simulink model "gnc_CommandShaping"  (R2026b)
settings: Solver=VariableStepAuto
values from neighbouring files (symbols this model uses):
  Ts = prm.Ts    [gnc_missionFSM.m]    (also in gnc_mpcPlantUpdate.m)
undefined symbols (not defined in the file or in its folder): accel_limit, beacon_cmd, buzzer_cmd, cmd_valid, gnc_ready, gnc_state, GncModeReq, mode_req, nav_fix, omega_cmd, P, seq, soft_stop_req, t_stamp, v_cmd, v_ground_est, v_ground_valid
libraries: simulink x4, sl_discontinuities x1
settings Model: Creator=aomar  LastModifiedBy=aomar

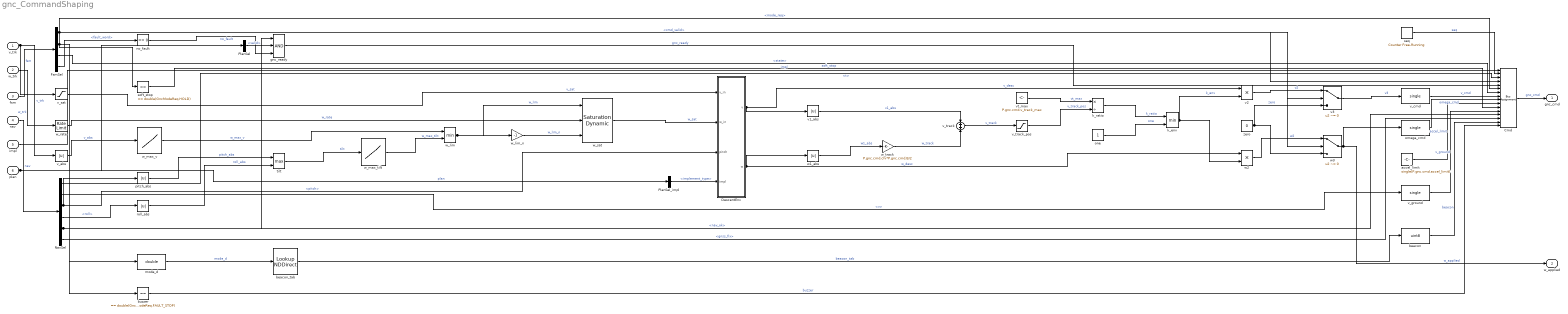
== system gnc_CommandShaping ==
  v_trk : Inport  OutDataTypeStr=double  PortDimensions=1  SampleTime=Ts.gnc
  w_trk : Inport  Port=2  OutDataTypeStr=double  PortDimensions=1  SampleTime=Ts.gnc
  fsm : Inport  Port=3  OutDataTypeStr=Bus: Bus_FsmOut  SampleTime=Ts.gnc
  nav : Inport  Port=4  OutDataTypeStr=Bus: Bus_NavCond  SampleTime=Ts.gnc
  impl : Inport  Port=5  OutDataTypeStr=Bus: Bus_GncCmd  SampleTime=Ts.gnc
  plan : Inport  Port=6  OutDataTypeStr=Bus: Bus_MissionPlan
  Cmd : BusAssignment  AssignedSignals=seq,t_stamp,cmd_valid,gnc_ready,mode_req,gnc_state,v_cmd,omega_cmd,accel_limit,soft_stop_req,v_ground_est,v_ground_valid,nav_fix,beacon_cmd,buzzer_cmd
  DescentEnv : MATLAB Function  TreatAsAtomicUnit=on  mask{desc=P.gnc.desc}
  FsmSel : BusSelector  OutputSignals=cmd_valid,mode_req,state,fault_word
  NavSel : BusSelector  OutputSignals=t,v,pitch,roll,nav_ok,gnss_fix
  PlanSel : BusSelector  OutputSignals=valid
  PlanSel_impl : BusSelector  OutputSignals=implement_type
  accel_limit : Constant  Value=single(P.gnc.cmd.accel_limit)  OutDataTypeStr=single  SampleTime=Ts.gnc
  beacon : DataTypeConversion  OutDataTypeStr=uint8  RndMeth=Nearest
  beacon_tab : LookupNDDirect  NumberOfTableDimensions=1  Table=P.gnc.cmd.beacon_by_mode  DiagnosticForOutOfRangeInput=None
  buzzer : simulink/Logic and Bit Operations/Compare To Constant  relop===  const=double(GncModeReq.FAULT_STOP)  OutDataTypeStr=boolean
  gnc_ready : Logic  Inputs=3  AllPortsSameDT=off  OutDataTypeStr=boolean
  k_env : MinMax  Inputs=2
  k_ratio : Product  Inputs=*/
  mode_d : DataTypeConversion  OutDataTypeStr=double  RndMeth=Nearest
  no_fault : simulink/Logic and Bit Operations/Compare To Constant  relop===  const=0  OutDataTypeStr=boolean
  omega_cmd : DataTypeConversion  OutDataTypeStr=single  RndMeth=Nearest
  one : Constant  OutDataTypeStr=double  SampleTime=Ts.gnc
  pitch_abs : Abs  SaturateOnIntegerOverflow=off
  roll_abs : Abs  SaturateOnIntegerOverflow=off
  seq : simulink/Sources/Counter Free-Running  NumBits=8  tsamp=Ts.gnc
  soft_stop : simulink/Logic and Bit Operations/Compare To Constant  relop===  const=double(GncModeReq.HOLD)  OutDataTypeStr=boolean
  tilt : MinMax  Function=max  Inputs=2
  v1_abs : Abs  SaturateOnIntegerOverflow=off
  v2 : Product  Inputs=**
  v3 : Switch  Criteria=u2 ~= 0  SaturateOnIntegerOverflow=off  InputSameDT=off
  v_abs : Abs  SaturateOnIntegerOverflow=off
  v_cmd : DataTypeConversion  OutDataTypeStr=single  RndMeth=Nearest
  v_ground : DataTypeConversion  OutDataTypeStr=single  RndMeth=Nearest
  v_sat : Saturate  UpperLimit=P.gnc.spd.v_max  LowerLimit=P.gnc.cmd.v_min_reverse
  v_track : Sum
  v_track_pos : Saturate  UpperLimit=inf  LowerLimit=1e-6
  vt_max : Constant  Value=P.gnc.cmd.v_track_max  OutDataTypeStr=double  SampleTime=Ts.gnc
  w1_abs : Abs  SaturateOnIntegerOverflow=off
  w2 : Product  Inputs=**
  w3 : Switch  Criteria=u2 ~= 0  SaturateOnIntegerOverflow=off  InputSameDT=off
  w_lim : MinMax  Inputs=2
  w_lim_n : Gain  Gain=-1
  w_max_tilt : Lookup_n-D  NumberOfTableDimensions=1  BreakpointsForDimension1=P.gnc.cmd.w_tilt_x  Table=P.gnc.cmd.w_tilt  ExtrapMethod=Clip  UseLastTableValue=on  InternalRulePriority=Speed  RndMeth=Simplest
  w_max_v : Lookup_n-D  NumberOfTableDimensions=1  BreakpointsForDimension1=P.gnc.cmd.w_max_v  Table=P.gnc.cmd.w_max  ExtrapMethod=Clip  UseLastTableValue=on  InternalRulePriority=Speed  RndMeth=Simplest
  w_rate : RateLimiter  RisingSlewLimit=P.gnc.cmd.w_rate  FallingSlewLimit=-P.gnc.cmd.w_rate  SampleTimeMode=inherited
  w_sat : sl_discontinuities/Saturation Dynamic  OutMin=[]  OutMax=[]  OutDataTypeStr=Inherit: Same as second input  OutDataType=fixdt(1, 16)  OutScaling=2^-10  DoSatur=off
      settings: LibrarySourceBlock=|
      | simulink/Discontinuities/Saturation
      | Dynamic
  w_track : Gain  Gain=P.gnc.cmd.chi*P.gnc.cmd.B/2
  zero : Constant  Value=0  OutDataTypeStr=double  SampleTime=Ts.gnc
  gnc_cmd : Outport  OutDataTypeStr=Bus: Bus_GncCmd
  w_applied : Outport  Port=2  OutDataTypeStr=double
  wires:
  v_trk/1 -> v_abs/1, v_sat/1  "v_trk"
  w_trk/1 -> w_rate/1  "w_trk"
  fsm/1 -> FsmSel/1  "fsm"
  nav/1 -> NavSel/1  "nav"
  impl/1 -> Cmd/1  "impl"
  plan/1 -> PlanSel/1, PlanSel_impl/1  "plan"
  FsmSel/1 -> w3/2, v3/2, Cmd/4  "<cmd_valid>"
  FsmSel/3 -> Cmd/7  "<state>"
  NavSel/1 -> Cmd/3  "<t>"
  NavSel/2 -> v_ground/1  "<v>"
  NavSel/3 -> DescentEnv/3(pitch), pitch_abs/1  "<pitch>"
  NavSel/4 -> roll_abs/1  "<roll>"
  NavSel/5 -> gnc_ready/1, Cmd/13  "<nav_ok>"
  NavSel/6 -> Cmd/14  "<gnss_fix>"
  v_sat/1 -> DescentEnv/1(v_in)  "v_sat"
  w_rate/1 -> w_sat/2  "w_rate"
  v_abs/1 -> w_max_v/1  "v_abs"
  no_fault/1 -> gnc_ready/3  "no_fault"
  soft_stop/1 -> Cmd/11  "soft_stop"
  pitch_abs/1 -> tilt/1  "pitch_abs"
  roll_abs/1 -> tilt/2  "roll_abs"
  buzzer/1 -> Cmd/16  "buzzer"
  w_max_v/1 -> w_lim/1  "w_max_v"
  mode_d/1 -> beacon_tab/1  "mode_d"
  PlanSel/1 -> gnc_ready/2  "<valid>"
  gnc_ready/1 -> Cmd/5  "gnc_ready"
  tilt/1 -> w_max_tilt/1  "tilt"
  beacon_tab/1 -> beacon/1  "beacon_tab"
  w_max_tilt/1 -> w_lim/2  "w_max_tilt"
  w_lim/1 -> w_sat/1, w_lim_n/1  "w_lim"
  w_lim_n/1 -> w_sat/3  "w_lim_n"
  w_sat/1 -> DescentEnv/2(w_in)  "w_sat"
  PlanSel_impl/1 -> DescentEnv/4(impl)  "<implement_type>"
  DescentEnv/1(v) -> v2/1, v1_abs/1  "v_desc"
  DescentEnv/2(w) -> w2/1, w1_abs/1  "w_desc"
  v1_abs/1 -> v_track/1  "v1_abs"
  w1_abs/1 -> w_track/1  "w1_abs"
  w_track/1 -> v_track/2  "w_track"
  v_track/1 -> v_track_pos/1  "v_track"
  vt_max/1 -> k_ratio/1  "vt_max"
  v_track_pos/1 -> k_ratio/2  "v_track_pos"
  k_ratio/1 -> k_env/1  "k_ratio"
  one/1 -> k_env/2  "one"
  k_env/1 -> w2/2, v2/2  "k_env"
  v2/1 -> v3/1  "v2"
  zero/1 -> w3/3, v3/3  "zero"
  w2/1 -> w3/1  "w2"
  v3/1 -> v_cmd/1  "v3"
  w3/1 -> w_applied/1, omega_cmd/1  "w_applied"
  seq/1 -> Cmd/2  "seq"
  accel_limit/1 -> Cmd/10  "accel_limit"
  v_cmd/1 -> Cmd/8  "v_cmd"
  omega_cmd/1 -> Cmd/9  "omega_cmd"
  v_ground/1 -> Cmd/12  "v_ground"
  beacon/1 -> Cmd/15  "beacon"
  Cmd/1 -> gnc_cmd/1  "gnc_cmd"
  FsmSel/2 -> buzzer/1, mode_d/1, Cmd/6, soft_stop/1  "<mode_req>"
  FsmSel/4 -> no_fault/1  "<fault_word>"

== matlab function gnc_CommandShaping/DescentEnv ==
  settings: updateMethod=DISCRETE  sampleTime=Ts.gnc  description=Downhill speed cap at the nav pitch, forward and reverse, omega scaled with v; body subsystems/gnc/gnc_descentEnvelope.m.
  data: v_in input; v output double; w_in input; pitch input; impl input; w output double; desc parameter
function [v, w] = fcn(v_in, w_in, pitch, impl, desc)
%#codegen
[v, w] = gnc_descentEnvelope(v_in, w_in, pitch, impl, desc);
